simulink model "sst_cllc_dcx"  (R2026b)
settings: Solver=ode23tb  StopTime=param.sim.simlength  FixedStep=tc  MaxStep=param.glb_time.tc
values from neighbouring files (symbols this model uses):
  param = struct()    [init_model.m]
undefined symbols (not defined in the file or in its folder): cllc_dcx_param_example
libraries: fl_lib x144, nesl_utility x71, mos_simple_2th_lib x8, discrete_time_low_pass_filter x2, lithium_ion_battery x1, cllc_dcx x1, single_phase_transformer x1, dab_single_phase_pwm_modulator x1, ee_lib x1
(part 4 of 4)

== system sst_cllc_dcx/dcdc_cllc_modA/dc//dc with galvanic isolation/full-bridge 1/full-full_bridge_ssc_mosfet_based/full_bridge_ssc_mosfet_based/mosfet_thermal_4/mos_simple_2th ==
  PS Terminator{,1..3} (4 alike) : fl_lib/Physical Signals/Sinks/PS Terminator
  mos_simple_2th : mos_simple_2th_lib/MOS_SIMPLE_2TH Simplified power MOSFET + antiparallel diode, two thermal ports  Rds_on=Rds_on_m Ohm  alpha_R=0 1/K  Tj_ref=398.15 K  Roff=1e7 Ohm  Vf=Vdon_diode_m V  Rd=Rdon_diode_m Ohm  two_die=1  G_th=0.5  Eon_ref=Eon_m J  Eoff_ref=Eoff_m J  Err_ref=0.5e-3 J  Iref=Ion_sw_loss_m A  Vref=Voff_sw_loss_m V  ki=1  kv=1  Vth_off=50 V  Vth_on=25 V  V_sm=10 V  tau_s=100e-9 s  tau_v=10e-6 s  tau_p=50e-6 s  i_eps=1e-3 A  v_eps=1e-3 V  v_specify=off  v_priority=None  v=0 V  v_nominal_specify=off  v_nominal_value=1  v_nominal_unit=V  i_specify=off  i_priority=None  i=0 A  i_nominal_specify=off  i_nominal_value=1  i_nominal_unit=A  ich_specify=off  ich_priority=None  ich=0 A  ich_nominal_specify=off  ich_nominal_value=1  ich_nominal_unit=A  ichp_specify=off  ichp_priority=None  ichp=0 A  ichp_nominal_specify=off  ichp_nominal_value=1  ichp_nominal_unit=A  idio_specify=off  idio_priority=None  idio=0 A  idio_nominal_specify=off  idio_nominal_value=1  idio_nominal_unit=A  vfd_specify=off  vfd_priority=None  vfd=0 V  vfd_nominal_specify=off  vfd_nominal_value=1  vfd_nominal_unit=V  ith_specify=off  ith_priority=None  ith=0 A  ith_nominal_specify=off  ith_nominal_value=1  ith_nominal_unit=A  idh_specify=off  idh_priority=None  idh=0 A  idh_nominal_specify=off  idh_nominal_value=1  idh_nominal_unit=A  vbl_specify=off  vbl_priority=None  vbl=600 V  vbl_nominal_specify=off  vbl_nominal_value=1  vbl_nominal_unit=V  hb_specify=off  hb_priority=None  hb=0  hb_nominal_specify=off  hb_nominal_value=1  hb_nominal_unit=1  Gch_specify=off  Gch_priority=None  Gch=0 S  Gch_nominal_specify=off  Gch_nominal_value=1  Gch_nominal_unit=S  gl_specify=off  gl_priority=None  gl=0  gl_nominal_specify=off  gl_nominal_value=1  gl_nominal_unit=1  Rds_specify=off  Rds_priority=None  Rds=1e-3 Ohm  Rds_nominal_specify=off  Rds_nominal_value=1  Rds_nominal_unit=Ohm  xr_specify=off  xr_priority=None  xr=1  xr_nominal_specify=off  xr_nominal_value=1  xr_nominal_unit=1  Eot_specify=off  Eot_priority=None  Eot=0 J  Eot_nominal_specify=off  Eot_nominal_value=1  Eot_nominal_unit=J  Eod_specify=off  Eod_priority=None  Eod=0 J  Eod_nominal_specify=off  Eod_nominal_value=1  Eod_nominal_unit=J  Pswt_specify=off  Pswt_priority=None  Pswt=0 W  Pswt_nominal_specify=off  Pswt_nominal_value=1  Pswt_nominal_unit=W  Pswd_specify=off  Pswd_priority=None  Pswd=0 W  Pswd_nominal_specify=off  Pswd_nominal_value=1  Pswd_nominal_unit=W  Pct_specify=off  Pct_priority=None  Pct=0 W  Pct_nominal_specify=off  Pct_nominal_value=1  Pct_nominal_unit=W  Pcd_specify=off  Pcd_priority=None  Pcd=0 W  Pcd_nominal_specify=off  Pcd_nominal_value=1  Pcd_nominal_unit=W  Qt_specify=off  Qt_priority=None  Qt=0 W  Qt_nominal_specify=off  Qt_nominal_value=1  Qt_nominal_unit=W  Qd_specify=off  Qd_priority=None  Qd=0 W  Qd_nominal_specify=off  Qd_nominal_value=1  Qd_nominal_unit=W  Eqt_specify=off  Eqt_priority=None  Eqt=0 J  Eqd_specify=off  Eqd_priority=None  Eqd=0 J
  G : PMIOPort  Side=Left
  H : PMIOPort  Port=2  Side=Left
  D : PMIOPort  Port=3  Side=Left
  S : PMIOPort  Port=4  Side=Right
  connections:
  mos_simple_2th/LConn1 -- D/RConn1
  mos_simple_2th/RConn1 -- S/RConn1
  mos_simple_2th/LConn3 -- G/RConn1
  mos_simple_2th/LConn2 -- mos_simple_2th/RConn2 -- H/RConn1
  PS Terminator/LConn1 -- mos_simple_2th/RConn3
  PS Terminator1/LConn1 -- mos_simple_2th/RConn4
  PS Terminator2/LConn1 -- mos_simple_2th/RConn5
  PS Terminator3/LConn1 -- mos_simple_2th/RConn6

== system sst_cllc_dcx/dcdc_cllc_modA/dc//dc with galvanic isolation/full-bridge 2/full_bridge_ssc_mosfet_based/full_bridge_ssc_mosfet_based/mosfet_thermal_1/mos_simple_2th ==
  PS Terminator{,1..3} (4 alike) : fl_lib/Physical Signals/Sinks/PS Terminator
  mos_simple_2th : mos_simple_2th_lib/MOS_SIMPLE_2TH Simplified power MOSFET + antiparallel diode, two thermal ports  Rds_on=Rds_on_m Ohm  alpha_R=0 1/K  Tj_ref=398.15 K  Roff=1e7 Ohm  Vf=Vdon_diode_m V  Rd=Rdon_diode_m Ohm  two_die=1  G_th=0.5  Eon_ref=Eon_m J  Eoff_ref=Eoff_m J  Err_ref=0.5e-3 J  Iref=Ion_sw_loss_m A  Vref=Voff_sw_loss_m V  ki=1  kv=1  Vth_off=50 V  Vth_on=25 V  V_sm=10 V  tau_s=100e-9 s  tau_v=10e-6 s  tau_p=50e-6 s  i_eps=1e-3 A  v_eps=1e-3 V  v_specify=off  v_priority=None  v=0 V  v_nominal_specify=off  v_nominal_value=1  v_nominal_unit=V  i_specify=off  i_priority=None  i=0 A  i_nominal_specify=off  i_nominal_value=1  i_nominal_unit=A  ich_specify=off  ich_priority=None  ich=0 A  ich_nominal_specify=off  ich_nominal_value=1  ich_nominal_unit=A  ichp_specify=off  ichp_priority=None  ichp=0 A  ichp_nominal_specify=off  ichp_nominal_value=1  ichp_nominal_unit=A  idio_specify=off  idio_priority=None  idio=0 A  idio_nominal_specify=off  idio_nominal_value=1  idio_nominal_unit=A  vfd_specify=off  vfd_priority=None  vfd=0 V  vfd_nominal_specify=off  vfd_nominal_value=1  vfd_nominal_unit=V  ith_specify=off  ith_priority=None  ith=0 A  ith_nominal_specify=off  ith_nominal_value=1  ith_nominal_unit=A  idh_specify=off  idh_priority=None  idh=0 A  idh_nominal_specify=off  idh_nominal_value=1  idh_nominal_unit=A  vbl_specify=off  vbl_priority=None  vbl=600 V  vbl_nominal_specify=off  vbl_nominal_value=1  vbl_nominal_unit=V  hb_specify=off  hb_priority=None  hb=0  hb_nominal_specify=off  hb_nominal_value=1  hb_nominal_unit=1  Gch_specify=off  Gch_priority=None  Gch=0 S  Gch_nominal_specify=off  Gch_nominal_value=1  Gch_nominal_unit=S  gl_specify=off  gl_priority=None  gl=0  gl_nominal_specify=off  gl_nominal_value=1  gl_nominal_unit=1  Rds_specify=off  Rds_priority=None  Rds=1e-3 Ohm  Rds_nominal_specify=off  Rds_nominal_value=1  Rds_nominal_unit=Ohm  xr_specify=off  xr_priority=None  xr=1  xr_nominal_specify=off  xr_nominal_value=1  xr_nominal_unit=1  Eot_specify=off  Eot_priority=None  Eot=0 J  Eot_nominal_specify=off  Eot_nominal_value=1  Eot_nominal_unit=J  Eod_specify=off  Eod_priority=None  Eod=0 J  Eod_nominal_specify=off  Eod_nominal_value=1  Eod_nominal_unit=J  Pswt_specify=off  Pswt_priority=None  Pswt=0 W  Pswt_nominal_specify=off  Pswt_nominal_value=1  Pswt_nominal_unit=W  Pswd_specify=off  Pswd_priority=None  Pswd=0 W  Pswd_nominal_specify=off  Pswd_nominal_value=1  Pswd_nominal_unit=W  Pct_specify=off  Pct_priority=None  Pct=0 W  Pct_nominal_specify=off  Pct_nominal_value=1  Pct_nominal_unit=W  Pcd_specify=off  Pcd_priority=None  Pcd=0 W  Pcd_nominal_specify=off  Pcd_nominal_value=1  Pcd_nominal_unit=W  Qt_specify=off  Qt_priority=None  Qt=0 W  Qt_nominal_specify=off  Qt_nominal_value=1  Qt_nominal_unit=W  Qd_specify=off  Qd_priority=None  Qd=0 W  Qd_nominal_specify=off  Qd_nominal_value=1  Qd_nominal_unit=W  Eqt_specify=off  Eqt_priority=None  Eqt=0 J  Eqd_specify=off  Eqd_priority=None  Eqd=0 J
  G : PMIOPort  Side=Left
  H : PMIOPort  Port=2  Side=Left
  D : PMIOPort  Port=3  Side=Left
  S : PMIOPort  Port=4  Side=Right
  connections:
  mos_simple_2th/LConn1 -- D/RConn1
  mos_simple_2th/RConn1 -- S/RConn1
  mos_simple_2th/LConn3 -- G/RConn1
  mos_simple_2th/LConn2 -- mos_simple_2th/RConn2 -- H/RConn1
  PS Terminator/LConn1 -- mos_simple_2th/RConn3
  PS Terminator1/LConn1 -- mos_simple_2th/RConn4
  PS Terminator2/LConn1 -- mos_simple_2th/RConn5
  PS Terminator3/LConn1 -- mos_simple_2th/RConn6

== system sst_cllc_dcx/dcdc_cllc_modA/dc//dc with galvanic isolation/full-bridge 2/full_bridge_ssc_mosfet_based/full_bridge_ssc_mosfet_based/mosfet_thermal_2/mos_simple_2th ==
  PS Terminator{,1..3} (4 alike) : fl_lib/Physical Signals/Sinks/PS Terminator
  mos_simple_2th : mos_simple_2th_lib/MOS_SIMPLE_2TH Simplified power MOSFET + antiparallel diode, two thermal ports  Rds_on=Rds_on_m Ohm  alpha_R=0 1/K  Tj_ref=398.15 K  Roff=1e7 Ohm  Vf=Vdon_diode_m V  Rd=Rdon_diode_m Ohm  two_die=1  G_th=0.5  Eon_ref=Eon_m J  Eoff_ref=Eoff_m J  Err_ref=0.5e-3 J  Iref=Ion_sw_loss_m A  Vref=Voff_sw_loss_m V  ki=1  kv=1  Vth_off=50 V  Vth_on=25 V  V_sm=10 V  tau_s=100e-9 s  tau_v=10e-6 s  tau_p=50e-6 s  i_eps=1e-3 A  v_eps=1e-3 V  v_specify=off  v_priority=None  v=0 V  v_nominal_specify=off  v_nominal_value=1  v_nominal_unit=V  i_specify=off  i_priority=None  i=0 A  i_nominal_specify=off  i_nominal_value=1  i_nominal_unit=A  ich_specify=off  ich_priority=None  ich=0 A  ich_nominal_specify=off  ich_nominal_value=1  ich_nominal_unit=A  ichp_specify=off  ichp_priority=None  ichp=0 A  ichp_nominal_specify=off  ichp_nominal_value=1  ichp_nominal_unit=A  idio_specify=off  idio_priority=None  idio=0 A  idio_nominal_specify=off  idio_nominal_value=1  idio_nominal_unit=A  vfd_specify=off  vfd_priority=None  vfd=0 V  vfd_nominal_specify=off  vfd_nominal_value=1  vfd_nominal_unit=V  ith_specify=off  ith_priority=None  ith=0 A  ith_nominal_specify=off  ith_nominal_value=1  ith_nominal_unit=A  idh_specify=off  idh_priority=None  idh=0 A  idh_nominal_specify=off  idh_nominal_value=1  idh_nominal_unit=A  vbl_specify=off  vbl_priority=None  vbl=600 V  vbl_nominal_specify=off  vbl_nominal_value=1  vbl_nominal_unit=V  hb_specify=off  hb_priority=None  hb=0  hb_nominal_specify=off  hb_nominal_value=1  hb_nominal_unit=1  Gch_specify=off  Gch_priority=None  Gch=0 S  Gch_nominal_specify=off  Gch_nominal_value=1  Gch_nominal_unit=S  gl_specify=off  gl_priority=None  gl=0  gl_nominal_specify=off  gl_nominal_value=1  gl_nominal_unit=1  Rds_specify=off  Rds_priority=None  Rds=1e-3 Ohm  Rds_nominal_specify=off  Rds_nominal_value=1  Rds_nominal_unit=Ohm  xr_specify=off  xr_priority=None  xr=1  xr_nominal_specify=off  xr_nominal_value=1  xr_nominal_unit=1  Eot_specify=off  Eot_priority=None  Eot=0 J  Eot_nominal_specify=off  Eot_nominal_value=1  Eot_nominal_unit=J  Eod_specify=off  Eod_priority=None  Eod=0 J  Eod_nominal_specify=off  Eod_nominal_value=1  Eod_nominal_unit=J  Pswt_specify=off  Pswt_priority=None  Pswt=0 W  Pswt_nominal_specify=off  Pswt_nominal_value=1  Pswt_nominal_unit=W  Pswd_specify=off  Pswd_priority=None  Pswd=0 W  Pswd_nominal_specify=off  Pswd_nominal_value=1  Pswd_nominal_unit=W  Pct_specify=off  Pct_priority=None  Pct=0 W  Pct_nominal_specify=off  Pct_nominal_value=1  Pct_nominal_unit=W  Pcd_specify=off  Pcd_priority=None  Pcd=0 W  Pcd_nominal_specify=off  Pcd_nominal_value=1  Pcd_nominal_unit=W  Qt_specify=off  Qt_priority=None  Qt=0 W  Qt_nominal_specify=off  Qt_nominal_value=1  Qt_nominal_unit=W  Qd_specify=off  Qd_priority=None  Qd=0 W  Qd_nominal_specify=off  Qd_nominal_value=1  Qd_nominal_unit=W  Eqt_specify=off  Eqt_priority=None  Eqt=0 J  Eqd_specify=off  Eqd_priority=None  Eqd=0 J
  G : PMIOPort  Side=Left
  H : PMIOPort  Port=2  Side=Left
  D : PMIOPort  Port=3  Side=Left
  S : PMIOPort  Port=4  Side=Right
  connections:
  mos_simple_2th/LConn1 -- D/RConn1
  mos_simple_2th/RConn1 -- S/RConn1
  mos_simple_2th/LConn3 -- G/RConn1
  mos_simple_2th/LConn2 -- mos_simple_2th/RConn2 -- H/RConn1
  PS Terminator/LConn1 -- mos_simple_2th/RConn3
  PS Terminator1/LConn1 -- mos_simple_2th/RConn4
  PS Terminator2/LConn1 -- mos_simple_2th/RConn5
  PS Terminator3/LConn1 -- mos_simple_2th/RConn6

== system sst_cllc_dcx/dcdc_cllc_modA/dc//dc with galvanic isolation/full-bridge 2/full_bridge_ssc_mosfet_based/full_bridge_ssc_mosfet_based/mosfet_thermal_3/mos_simple_2th ==
  PS Terminator{,1..3} (4 alike) : fl_lib/Physical Signals/Sinks/PS Terminator
  mos_simple_2th : mos_simple_2th_lib/MOS_SIMPLE_2TH Simplified power MOSFET + antiparallel diode, two thermal ports  Rds_on=Rds_on_m Ohm  alpha_R=0 1/K  Tj_ref=398.15 K  Roff=1e7 Ohm  Vf=Vdon_diode_m V  Rd=Rdon_diode_m Ohm  two_die=1  G_th=0.5  Eon_ref=Eon_m J  Eoff_ref=Eoff_m J  Err_ref=0.5e-3 J  Iref=Ion_sw_loss_m A  Vref=Voff_sw_loss_m V  ki=1  kv=1  Vth_off=50 V  Vth_on=25 V  V_sm=10 V  tau_s=100e-9 s  tau_v=10e-6 s  tau_p=50e-6 s  i_eps=1e-3 A  v_eps=1e-3 V  v_specify=off  v_priority=None  v=0 V  v_nominal_specify=off  v_nominal_value=1  v_nominal_unit=V  i_specify=off  i_priority=None  i=0 A  i_nominal_specify=off  i_nominal_value=1  i_nominal_unit=A  ich_specify=off  ich_priority=None  ich=0 A  ich_nominal_specify=off  ich_nominal_value=1  ich_nominal_unit=A  ichp_specify=off  ichp_priority=None  ichp=0 A  ichp_nominal_specify=off  ichp_nominal_value=1  ichp_nominal_unit=A  idio_specify=off  idio_priority=None  idio=0 A  idio_nominal_specify=off  idio_nominal_value=1  idio_nominal_unit=A  vfd_specify=off  vfd_priority=None  vfd=0 V  vfd_nominal_specify=off  vfd_nominal_value=1  vfd_nominal_unit=V  ith_specify=off  ith_priority=None  ith=0 A  ith_nominal_specify=off  ith_nominal_value=1  ith_nominal_unit=A  idh_specify=off  idh_priority=None  idh=0 A  idh_nominal_specify=off  idh_nominal_value=1  idh_nominal_unit=A  vbl_specify=off  vbl_priority=None  vbl=600 V  vbl_nominal_specify=off  vbl_nominal_value=1  vbl_nominal_unit=V  hb_specify=off  hb_priority=None  hb=0  hb_nominal_specify=off  hb_nominal_value=1  hb_nominal_unit=1  Gch_specify=off  Gch_priority=None  Gch=0 S  Gch_nominal_specify=off  Gch_nominal_value=1  Gch_nominal_unit=S  gl_specify=off  gl_priority=None  gl=0  gl_nominal_specify=off  gl_nominal_value=1  gl_nominal_unit=1  Rds_specify=off  Rds_priority=None  Rds=1e-3 Ohm  Rds_nominal_specify=off  Rds_nominal_value=1  Rds_nominal_unit=Ohm  xr_specify=off  xr_priority=None  xr=1  xr_nominal_specify=off  xr_nominal_value=1  xr_nominal_unit=1  Eot_specify=off  Eot_priority=None  Eot=0 J  Eot_nominal_specify=off  Eot_nominal_value=1  Eot_nominal_unit=J  Eod_specify=off  Eod_priority=None  Eod=0 J  Eod_nominal_specify=off  Eod_nominal_value=1  Eod_nominal_unit=J  Pswt_specify=off  Pswt_priority=None  Pswt=0 W  Pswt_nominal_specify=off  Pswt_nominal_value=1  Pswt_nominal_unit=W  Pswd_specify=off  Pswd_priority=None  Pswd=0 W  Pswd_nominal_specify=off  Pswd_nominal_value=1  Pswd_nominal_unit=W  Pct_specify=off  Pct_priority=None  Pct=0 W  Pct_nominal_specify=off  Pct_nominal_value=1  Pct_nominal_unit=W  Pcd_specify=off  Pcd_priority=None  Pcd=0 W  Pcd_nominal_specify=off  Pcd_nominal_value=1  Pcd_nominal_unit=W  Qt_specify=off  Qt_priority=None  Qt=0 W  Qt_nominal_specify=off  Qt_nominal_value=1  Qt_nominal_unit=W  Qd_specify=off  Qd_priority=None  Qd=0 W  Qd_nominal_specify=off  Qd_nominal_value=1  Qd_nominal_unit=W  Eqt_specify=off  Eqt_priority=None  Eqt=0 J  Eqd_specify=off  Eqd_priority=None  Eqd=0 J
  G : PMIOPort  Side=Left
  H : PMIOPort  Port=2  Side=Left
  D : PMIOPort  Port=3  Side=Left
  S : PMIOPort  Port=4  Side=Right
  connections:
  mos_simple_2th/LConn1 -- D/RConn1
  mos_simple_2th/RConn1 -- S/RConn1
  mos_simple_2th/LConn3 -- G/RConn1
  mos_simple_2th/LConn2 -- mos_simple_2th/RConn2 -- H/RConn1
  PS Terminator/LConn1 -- mos_simple_2th/RConn3
  PS Terminator1/LConn1 -- mos_simple_2th/RConn4
  PS Terminator2/LConn1 -- mos_simple_2th/RConn5
  PS Terminator3/LConn1 -- mos_simple_2th/RConn6

== system sst_cllc_dcx/dcdc_cllc_modA/dc//dc with galvanic isolation/full-bridge 2/full_bridge_ssc_mosfet_based/full_bridge_ssc_mosfet_based/mosfet_thermal_4/mos_simple_2th ==
  PS Terminator{,1..3} (4 alike) : fl_lib/Physical Signals/Sinks/PS Terminator
  mos_simple_2th : mos_simple_2th_lib/MOS_SIMPLE_2TH Simplified power MOSFET + antiparallel diode, two thermal ports  Rds_on=Rds_on_m Ohm  alpha_R=0 1/K  Tj_ref=398.15 K  Roff=1e7 Ohm  Vf=Vdon_diode_m V  Rd=Rdon_diode_m Ohm  two_die=1  G_th=0.5  Eon_ref=Eon_m J  Eoff_ref=Eoff_m J  Err_ref=0.5e-3 J  Iref=Ion_sw_loss_m A  Vref=Voff_sw_loss_m V  ki=1  kv=1  Vth_off=50 V  Vth_on=25 V  V_sm=10 V  tau_s=100e-9 s  tau_v=10e-6 s  tau_p=50e-6 s  i_eps=1e-3 A  v_eps=1e-3 V  v_specify=off  v_priority=None  v=0 V  v_nominal_specify=off  v_nominal_value=1  v_nominal_unit=V  i_specify=off  i_priority=None  i=0 A  i_nominal_specify=off  i_nominal_value=1  i_nominal_unit=A  ich_specify=off  ich_priority=None  ich=0 A  ich_nominal_specify=off  ich_nominal_value=1  ich_nominal_unit=A  ichp_specify=off  ichp_priority=None  ichp=0 A  ichp_nominal_specify=off  ichp_nominal_value=1  ichp_nominal_unit=A  idio_specify=off  idio_priority=None  idio=0 A  idio_nominal_specify=off  idio_nominal_value=1  idio_nominal_unit=A  vfd_specify=off  vfd_priority=None  vfd=0 V  vfd_nominal_specify=off  vfd_nominal_value=1  vfd_nominal_unit=V  ith_specify=off  ith_priority=None  ith=0 A  ith_nominal_specify=off  ith_nominal_value=1  ith_nominal_unit=A  idh_specify=off  idh_priority=None  idh=0 A  idh_nominal_specify=off  idh_nominal_value=1  idh_nominal_unit=A  vbl_specify=off  vbl_priority=None  vbl=600 V  vbl_nominal_specify=off  vbl_nominal_value=1  vbl_nominal_unit=V  hb_specify=off  hb_priority=None  hb=0  hb_nominal_specify=off  hb_nominal_value=1  hb_nominal_unit=1  Gch_specify=off  Gch_priority=None  Gch=0 S  Gch_nominal_specify=off  Gch_nominal_value=1  Gch_nominal_unit=S  gl_specify=off  gl_priority=None  gl=0  gl_nominal_specify=off  gl_nominal_value=1  gl_nominal_unit=1  Rds_specify=off  Rds_priority=None  Rds=1e-3 Ohm  Rds_nominal_specify=off  Rds_nominal_value=1  Rds_nominal_unit=Ohm  xr_specify=off  xr_priority=None  xr=1  xr_nominal_specify=off  xr_nominal_value=1  xr_nominal_unit=1  Eot_specify=off  Eot_priority=None  Eot=0 J  Eot_nominal_specify=off  Eot_nominal_value=1  Eot_nominal_unit=J  Eod_specify=off  Eod_priority=None  Eod=0 J  Eod_nominal_specify=off  Eod_nominal_value=1  Eod_nominal_unit=J  Pswt_specify=off  Pswt_priority=None  Pswt=0 W  Pswt_nominal_specify=off  Pswt_nominal_value=1  Pswt_nominal_unit=W  Pswd_specify=off  Pswd_priority=None  Pswd=0 W  Pswd_nominal_specify=off  Pswd_nominal_value=1  Pswd_nominal_unit=W  Pct_specify=off  Pct_priority=None  Pct=0 W  Pct_nominal_specify=off  Pct_nominal_value=1  Pct_nominal_unit=W  Pcd_specify=off  Pcd_priority=None  Pcd=0 W  Pcd_nominal_specify=off  Pcd_nominal_value=1  Pcd_nominal_unit=W  Qt_specify=off  Qt_priority=None  Qt=0 W  Qt_nominal_specify=off  Qt_nominal_value=1  Qt_nominal_unit=W  Qd_specify=off  Qd_priority=None  Qd=0 W  Qd_nominal_specify=off  Qd_nominal_value=1  Qd_nominal_unit=W  Eqt_specify=off  Eqt_priority=None  Eqt=0 J  Eqd_specify=off  Eqd_priority=None  Eqd=0 J
  G : PMIOPort  Side=Left
  H : PMIOPort  Port=2  Side=Left
  D : PMIOPort  Port=3  Side=Left
  S : PMIOPort  Port=4  Side=Right
  connections:
  mos_simple_2th/LConn1 -- D/RConn1
  mos_simple_2th/RConn1 -- S/RConn1
  mos_simple_2th/LConn3 -- G/RConn1
  mos_simple_2th/LConn2 -- mos_simple_2th/RConn2 -- H/RConn1
  PS Terminator/LConn1 -- mos_simple_2th/RConn3
  PS Terminator1/LConn1 -- mos_simple_2th/RConn4
  PS Terminator2/LConn1 -- mos_simple_2th/RConn5
  PS Terminator3/LConn1 -- mos_simple_2th/RConn6
